simulink model "CombinedExperiment"  (R2020a)
settings: Solver=FixedStepAuto  StartTime=0.0  StopTime=tsim  FixedStep=baseRate  RelTol=1e-3  EnableMultiTasking=on
values from neighbouring files (symbols this model uses):
  baseRate = 0.1    [Run_Initializer.m]
  drop_states_BLACK = [1.36947387695313,1.22175756835938,-0.0161599479615688]    [Run_Initializer.m]
  drop_states_BLUE = [ xLength/2+0.9; yLength/2+0.5; 0]    [Run_Initializer.m]
  drop_states_RED = [ xLength/2+1.1; yLength/2; pi]    [Run_Initializer.m]
  F_thrusters_BLACK = 0.25.*ones(8,1)    [Run_Initializer.m]
  F_thrusters_BLUE = 0.25.*ones(8,1)    [Run_Initializer.m]
  F_thrusters_RED = 0.25.*ones(8,1)    [Run_Initializer.m]
  home_states_BLACK = [ xLength/2; yLength/2; 0]    [Run_Initializer.m]
  home_states_BLUE = [ xLength/2-0.9; yLength/2+0.5; 0]    [Run_Initializer.m]
  home_states_RED = [ xLength/2+1.1; yLength/2; pi]    [Run_Initializer.m]
  init_states_BLACK = [ xLength/2; yLength/2; 0]    [Run_Initializer.m]
  init_states_BLUE = [ xLength/2+0.9; yLength/2+0.5; 0]    [Run_Initializer.m]
  init_states_RED = [ xLength/2+1.1; yLength/2; pi]    [Run_Initializer.m]
  Kd_tb = 0.4    [Run_Initializer.m]
  Kd_tblue = 0.4    [Run_Initializer.m]
  Kd_tr = 0.4    [Run_Initializer.m]
  Kd_xb = 5    [Run_Initializer.m]
  Kd_xblue = 5    [Run_Initializer.m]
  Kd_xr = 5    [Run_Initializer.m]
  Kd_yb = 5    [Run_Initializer.m]
  Kd_yblue = 5    [Run_Initializer.m]
  Kd_yr = 5    [Run_Initializer.m]
  Kp_tb = 0.1    [Run_Initializer.m]
  Kp_tblue = 0.1    [Run_Initializer.m]
  Kp_tr = 0.1    [Run_Initializer.m]
  Kp_xb = 2    [Run_Initializer.m]
  Kp_xblue = 2    [Run_Initializer.m]
  Kp_xr = 2    [Run_Initializer.m]
  Kp_yb = 2    [Run_Initializer.m]
  Kp_yblue = 2    [Run_Initializer.m]
  Kp_yr = 2    [Run_Initializer.m]
  noise_variance_BLACK = 0    [Run_Initializer.m]
  noise_variance_BLUE = 0    [Run_Initializer.m]
  noise_variance_RED = 0    [Run_Initializer.m]
  Phase0_End = Phase0_Duration    (= 10)    [Run_Initializer.m]
  Phase1_End = Phase0_Duration + Phase1_Duration    (= 15)    [Run_Initializer.m]
  Phase2_End = Phase0_Duration + Phase1_Duration +                                   Phase2_Duration    (= 40)    [Run_Initializer.m]
  Phase3_End = Phase0_Duration + Phase1_Duration +                                   Phase2_Duration + Phase3_Duration    (= 117)    [Run_Initializer.m]
  Phase3_SubPhase1_End = Phase2_End + Phase3_SubPhase1_Duration    (= 41)    [Run_Initializer.m]
  Phase3_SubPhase2_End = Phase2_End + Phase3_SubPhase1_Duration +                                   Phase3_SubPhase2_Duration    (= 42)    [Run_Initializer.m]
  Phase3_SubPhase3_End = Phase2_End + Phase3_SubPhase1_Duration +                                   Phase3_SubPhase2_Duration +                                  Phase3_SubPhase3_Duration    (= 72)    [Run_Initializer.m]
  Phase3_SubPhase4_End = Phase2_End + Phase3_SubPhase1_Duration +                                   Phase3_SubPhase2_Duration +                                  Phase3_SubPhase3_Duration +                                  Phase3_SubPhase4_Duration    [Run_Initializer.m]
  Phase4_End = Phase0_Duration + Phase1_Duration +                                   Phase2_Duration + Phase3_Duration +                                   Phase4_Duration    (= 137)    [Run_Initializer.m]
  Phase5_End = Phase0_Duration + Phase1_Duration +                                   Phase2_Duration + Phase3_Duration +                                   Phase4_Duration + Phase5_Duration    (= 142)    [Run_Initializer.m]
  serverRate = 0.2    [Run_Initializer.m]
  thruster_dist2CG_BLACK = [83.42;-52.58;55.94;-60.05;54.08;-53.92;77.06;-55.94]    [Run_Initializer.m]
  thruster_dist2CG_BLUE = [83.42;-52.58;55.94;-60.05;54.08;-53.92;77.06;-55.94]    [Run_Initializer.m]
  thruster_dist2CG_RED = [49.92;-78.08;70.46;-63.54;81.08;-50.42;57.44;-75.96]    [Run_Initializer.m]
  xLength = 3.51155    [Run_Initializer.m]
  yLength = 2.41935    [Run_Initializer.m]
undefined symbols (not defined in the file or in its folder): DiscIntNeverNeededParam, platformSelection, simMode, WhoAmI
libraries: dspstat3 x18, raspberrypiBasiclib x10, dspsigops x9, embdlinuxlib x8, simulink x8, MainLibrary x5, mspfiltlib x3, dsparch4 x3, dspswit3 x2, sensehatlib x1
(part 9 of 9)

== matlab function CombinedExperiment/From Force//Torque to PWM Signal/Change BLACK Behavior/Calculate Thruster ON//OFF/Rotate Forces to Inertial/Create Rotation Matrix ==
  data: Rz input; C_Ib output
function C_Ib = RotateFrame(Rz)

C_bI = [  cos(Rz) sin(Rz)
         -sin(Rz) cos(Rz) ];

C_Ib = inv(C_bI);

end

== matlab function CombinedExperiment/From Force//Torque to PWM Signal/Change BLACK Behavior/Rotate Forces to Body/Create Rotation Matrix ==
  data: Rz input; C_bI output
function C_bI = RotateFrame(Rz)

C_bI = [  cos(Rz) sin(Rz)
         -sin(Rz) cos(Rz) ];

end

== matlab function CombinedExperiment/From Force//Torque to PWM Signal/Change RED Behavior/Calculate Thruster ON//OFF/MATLAB Function ==
  data: H output; thruster_dist2CG_RED parameter; F_thrusters_RED parameter
function H = MakeH(thruster_dist2CG_RED,F_thrusters_RED)

Vec1 = [ -1
         -1
          0 
          0
          1
          1
          0
          0 ];
      
Vec2 = [  0
          0
          1
          1
          0
          0
         -1
         -1 ];
     
Vec3 = thruster_dist2CG_RED./1000;

Mat1 = [Vec1, Vec2, Vec3]';

Mat2 = diag((F_thrusters_RED./2));

H    = Mat1*Mat2;

end

== matlab function CombinedExperiment/From Force//Torque to PWM Signal/Change RED Behavior/Calculate Thruster ON//OFF/MATLAB Function1 ==
  data: H output; thruster_dist2CG_RED parameter; F_thrusters_RED parameter
function H = MakeH(thruster_dist2CG_RED,F_thrusters_RED)

Vec1 = [ -1
         -1
          0 
          0
          1
          1
          0
          0 ];
      
Vec2 = [  0
          0
          1
          1
          0
          0
         -1
         -1 ];
     
Vec3 = thruster_dist2CG_RED./1000;

Mat1 = [Vec1, Vec2, Vec3]';

Mat2 = diag((F_thrusters_RED));

H    = Mat1*Mat2;

end

== matlab function CombinedExperiment/From Force//Torque to PWM Signal/Change RED Behavior/Calculate Thruster ON//OFF/MATLAB Function2 ==
  data: ThrustPer_Final output; ThrustPer input
function ThrustPer_Final  = ThrusterSat(ThrustPer)

ValveTime       = 0.007;
TControl        = 0.1;
ThrustPer_Final = zeros(8,1);

if max(ThrustPer) > 1
    ThrustPer_Sat = ThrustPer/max(ThrustPer);
else
    ThrustPer_Sat = ThrustPer;
end

for i = 1:8
    if ThrustPer_Sat(i) > ValveTime/TControl 
        ThrustPer_Final(i) = ThrustPer_Sat(i);
    else
        ThrustPer_Final(i) = 0;
    end
end
   

end

== matlab function CombinedExperiment/Simulate Plant Dynamics/RED Dynamics Model/MATLAB Function ==
  data: control_inputs input; x_ddot output; model_param parameter
function x_ddot = RED_dynamics(control_inputs, model_param)

%#codegen
% Fully define the size of x_ddot() for code generation:
x_ddot     = zeros(3,1);

% Extract the servicer model parameters from the model_param vector defined
% in initialize.m:
m_RED    = model_param(1);
I_RED    = model_param(2);

% Extract the control inputs from the control_input vector:
Fx        = control_inputs(1);              % [N]
Fy        = control_inputs(2);              % [N]
Tz        = control_inputs(3);              % [N.m]

% Calculate the state acceleration vector:
x_ddot(1) = Fx/m_RED;                      % [m/s^2]
x_ddot(2) = Fy/m_RED;                      % [m/s^2]
x_ddot(3) = Tz/I_RED;                      % [rad/s^2]

end

== matlab function CombinedExperiment/From Force//Torque to PWM Signal/Change RED Behavior/Calculate Thruster ON//OFF/Rotate Forces to Inertial/Create Rotation Matrix ==
  data: Rz input; C_Ib output
function C_Ib = RotateFrame(Rz)

C_bI = [  cos(Rz) sin(Rz)
         -sin(Rz) cos(Rz) ];

C_Ib = inv(C_bI);

end

== matlab function CombinedExperiment/Simulate Plant Dynamics/Sample and Hold Data to Match PhaseSpace (RED)/MATLAB Function ==
  data: TIME input; y output; SERVER input
function y = fcn(TIME, SERVER)

if mod(TIME,SERVER) == 0
    y = 1;
else
    y = 0;
end

== matlab function CombinedExperiment/Simulate Plant Dynamics/Sample and Hold Data to Match PhaseSpace (BLACK)/MATLAB Function ==
  data: TIME input; y output; SERVER input
function y = fcn(TIME, SERVER)

if mod(TIME,SERVER) == 0
    y = 1;
else
    y = 0;
end

== matlab function CombinedExperiment/From Force//Torque to PWM Signal/Change RED Behavior/Rotate Forces to Body/Create Rotation Matrix ==
  data: Rz input; C_bI output
function C_bI = RotateFrame(Rz)

C_bI = [  cos(Rz) sin(Rz)
         -sin(Rz) cos(Rz) ];

end

== matlab function CombinedExperiment/Phase #2: Move to Initial Position/Change RED Behavior/Hough Control/MATLAB Function2 ==
  data: Oy output; z input; Ox output
function [Oy, Ox]   = C3( z )
%C3 gives the rotation matrix about the z-axis for an angle 'z'
%   z - the angle about the z-axis which you rotate
%   A - the rotation matrix

Ox = [cos(z) sin(z); -sin(z) cos(z)]*[1;0];
Oy = [cos(z) sin(z); -sin(z) cos(z)]*[0;1];
end

== matlab function CombinedExperiment/Phase #2: Move to Initial Position/Change RED Behavior/Hough Control/MATLAB Function3 ==
  data: z input; Ox output
function Ox    = C3( z )
%C3 gives the rotation matrix about the z-axis for an angle 'z'
%   z - the angle about the z-axis which you rotate
%   A - the rotation matrix

Ox = [cos(z) sin(z); -sin(z) cos(z)]*[1;0];
end

== matlab function CombinedExperiment/Phase #2: Move to Initial Position/Change RED Behavior/Hough Control/MATLAB Function4 ==
  data: Oy input; e_out output; e_in input
function e_out = fcn(Oy, e_in)

a = sign(Oy'*e_in);
e_out = -a*norm(e_in);

== matlab function CombinedExperiment/Phase #3: Experiment/Change BLACK Behavior/Sub-Phase #4/Hough Control/MATLAB Function3 ==
  data: z input; Ox output
function Ox    = C3( z )
%C3 gives the rotation matrix about the z-axis for an angle 'z'
%   z - the angle about the z-axis which you rotate
%   A - the rotation matrix

Ox = [cos(z) sin(z); -sin(z) cos(z)]*[1;0];
end

== matlab function CombinedExperiment/Phase #4: Return Home/Change BLACK Behavior/Hough Control/MATLAB Function2 ==
  data: Oy output; z input; Ox output
function [Oy, Ox]   = C3( z )
%C3 gives the rotation matrix about the z-axis for an angle 'z'
%   z - the angle about the z-axis which you rotate
%   A - the rotation matrix

Ox = [cos(z) sin(z); -sin(z) cos(z)]*[1;0];
Oy = [cos(z) sin(z); -sin(z) cos(z)]*[0;1];
end

== matlab function CombinedExperiment/Phase #4: Return Home/Change BLACK Behavior/Hough Control/MATLAB Function3 ==
  data: z input; Ox output
function Ox    = C3( z )
%C3 gives the rotation matrix about the z-axis for an angle 'z'
%   z - the angle about the z-axis which you rotate
%   A - the rotation matrix

Ox = [cos(z) sin(z); -sin(z) cos(z)]*[1;0];
end

== matlab function CombinedExperiment/Simulate Plant Dynamics/BLACK Dynamics Model/MATLAB Function ==
  data: control_inputs input; x_ddot output; model_param parameter
function x_ddot = BLACK_dynamics(control_inputs, model_param)

%#codegen
% Fully define the size of x_ddot() for code generation:
x_ddot     = zeros(3,1);

% Extract the servicer model parameters from the model_param vector defined
% in initialize.m:
m_BLACK    = model_param(3);
I_BLACK    = model_param(4);

% Extract the control inputs from the control_input vector:
Fx        = control_inputs(1);              % [N]
Fy        = control_inputs(2);              % [N]
Tz        = control_inputs(3);              % [N.m]

% Calculate the state acceleration vector:
x_ddot(1) = Fx/m_BLACK;                      % [m/s^2]
x_ddot(2) = Fy/m_BLACK;                      % [m/s^2]
x_ddot(3) = Tz/I_BLACK;                      % [rad/s^2]

end

== matlab function CombinedExperiment/Phase #4: Return Home/Change BLACK Behavior/Hough Control/MATLAB Function4 ==
  data: Oy input; e_out output; e_in input
function e_out = fcn(Oy, e_in)

a = sign(Oy'*e_in);
e_out = -a*norm(e_in);

== matlab function CombinedExperiment/Phase #4: Return Home/Change RED Behavior/Hough Control/MATLAB Function2 ==
  data: Oy output; z input; Ox output
function [Oy, Ox]   = C3( z )
%C3 gives the rotation matrix about the z-axis for an angle 'z'
%   z - the angle about the z-axis which you rotate
%   A - the rotation matrix

Ox = [cos(z) sin(z); -sin(z) cos(z)]*[1;0];
Oy = [cos(z) sin(z); -sin(z) cos(z)]*[0;1];
end

== matlab function CombinedExperiment/Phase #4: Return Home/Change RED Behavior/Hough Control/MATLAB Function3 ==
  data: z input; Ox output
function Ox    = C3( z )
%C3 gives the rotation matrix about the z-axis for an angle 'z'
%   z - the angle about the z-axis which you rotate
%   A - the rotation matrix

Ox = [cos(z) sin(z); -sin(z) cos(z)]*[1;0];
end

== matlab function CombinedExperiment/Phase #4: Return Home/Change RED Behavior/Hough Control/MATLAB Function4 ==
  data: Oy input; e_out output; e_in input
function e_out = fcn(Oy, e_in)

a = sign(Oy'*e_in);
e_out = -a*norm(e_in);

== matlab function CombinedExperiment/Phase #2: Move to Initial Position/Change BLUE Behavior/Hough Control/MATLAB Function2 ==
  data: Oy output; z input; Ox output
function [Oy, Ox]   = C3( z )
%C3 gives the rotation matrix about the z-axis for an angle 'z'
%   z - the angle about the z-axis which you rotate
%   A - the rotation matrix

Ox = [cos(z) sin(z); -sin(z) cos(z)]*[1;0];
Oy = [cos(z) sin(z); -sin(z) cos(z)]*[0;1];
end

== matlab function CombinedExperiment/Phase #2: Move to Initial Position/Change BLUE Behavior/Hough Control/MATLAB Function3 ==
  data: z input; Ox output
function Ox    = C3( z )
%C3 gives the rotation matrix about the z-axis for an angle 'z'
%   z - the angle about the z-axis which you rotate
%   A - the rotation matrix

Ox = [cos(z) sin(z); -sin(z) cos(z)]*[1;0];
end

== matlab function CombinedExperiment/Phase #2: Move to Initial Position/Change BLUE Behavior/Hough Control/MATLAB Function4 ==
  data: Oy input; e_out output; e_in input
function e_out = fcn(Oy, e_in)

a = sign(Oy'*e_in);
e_out = -a*norm(e_in);

== matlab function CombinedExperiment/Phase #3: Experiment/Change BLUE Behavior/Sub-Phase #1/Hough Control/MATLAB Function2 ==
  data: Oy output; z input; Ox output
function [Oy, Ox]   = C3( z )
%C3 gives the rotation matrix about the z-axis for an angle 'z'
%   z - the angle about the z-axis which you rotate
%   A - the rotation matrix

Ox = [cos(z) sin(z); -sin(z) cos(z)]*[1;0];
Oy = [cos(z) sin(z); -sin(z) cos(z)]*[0;1];
end

== matlab function CombinedExperiment/Phase #3: Experiment/Change RED Behavior/Sub-Phase #4/Hough Control1/MATLAB Function2 ==
  data: Oy output; z input; Ox output
function [Oy, Ox]   = C3( z )
%C3 gives the rotation matrix about the z-axis for an angle 'z'
%   z - the angle about the z-axis which you rotate
%   A - the rotation matrix

Ox = [cos(z) sin(z); -sin(z) cos(z)]*[1;0];
Oy = [cos(z) sin(z); -sin(z) cos(z)]*[0;1];
end

== matlab function CombinedExperiment/Phase #3: Experiment/Change RED Behavior/Sub-Phase #4/Hough Control1/MATLAB Function3 ==
  data: z input; Ox output
function Ox    = C3( z )
%C3 gives the rotation matrix about the z-axis for an angle 'z'
%   z - the angle about the z-axis which you rotate
%   A - the rotation matrix

Ox = [cos(z) sin(z); -sin(z) cos(z)]*[1;0];
end

== matlab function CombinedExperiment/Phase #3: Experiment/Change RED Behavior/Sub-Phase #4/Hough Control1/MATLAB Function4 ==
  data: Oy input; e_out output; e_in input
function e_out = fcn(Oy, e_in)

a = sign(Oy'*e_in);
e_out = -a*norm(e_in);

== matlab function CombinedExperiment/Simulate Plant Dynamics/Sample and Hold Data to Match PhaseSpace (BLUE)/MATLAB Function ==
  data: TIME input; y output; SERVER input
function y = fcn(TIME, SERVER)

if mod(TIME,SERVER) == 0
    y = 1;
else
    y = 0;
end

== matlab function CombinedExperiment/Phase #3: Experiment/Change BLUE Behavior/Sub-Phase #1/Hough Control/MATLAB Function3 ==
  data: z input; Ox output
function Ox    = C3( z )
%C3 gives the rotation matrix about the z-axis for an angle 'z'
%   z - the angle about the z-axis which you rotate
%   A - the rotation matrix

Ox = [cos(z) sin(z); -sin(z) cos(z)]*[1;0];
end

== matlab function CombinedExperiment/Phase #3: Experiment/Change BLUE Behavior/Sub-Phase #1/Hough Control/MATLAB Function4 ==
  data: Oy input; e_out output; e_in input
function e_out = fcn(Oy, e_in)

a = sign(Oy'*e_in);
e_out = -a*norm(e_in);

== matlab function CombinedExperiment/Phase #3: Experiment/Change BLUE Behavior/Sub-Phase #4/Hough Control/MATLAB Function2 ==
  data: Oy output; z input; Ox output
function [Oy, Ox]   = C3( z )
%C3 gives the rotation matrix about the z-axis for an angle 'z'
%   z - the angle about the z-axis which you rotate
%   A - the rotation matrix

Ox = [cos(z) sin(z); -sin(z) cos(z)]*[1;0];
Oy = [cos(z) sin(z); -sin(z) cos(z)]*[0;1];
end

== matlab function CombinedExperiment/Phase #3: Experiment/Change RED Behavior/Sub-Phase #4/Hough Control/MATLAB Function2 ==
  data: Oy output; z input; Ox output
function [Oy, Ox]   = C3( z )
%C3 gives the rotation matrix about the z-axis for an angle 'z'
%   z - the angle about the z-axis which you rotate
%   A - the rotation matrix

Ox = [cos(z) sin(z); -sin(z) cos(z)]*[1;0];
Oy = [cos(z) sin(z); -sin(z) cos(z)]*[0;1];
end

== matlab function CombinedExperiment/Phase #3: Experiment/Change RED Behavior/Sub-Phase #4/Hough Control/MATLAB Function3 ==
  data: z input; Ox output
function Ox    = C3( z )
%C3 gives the rotation matrix about the z-axis for an angle 'z'
%   z - the angle about the z-axis which you rotate
%   A - the rotation matrix

Ox = [cos(z) sin(z); -sin(z) cos(z)]*[1;0];
end

== matlab function CombinedExperiment/Phase #3: Experiment/Change RED Behavior/Sub-Phase #4/Hough Control/MATLAB Function4 ==
  data: Oy input; e_out output; e_in input
function e_out = fcn(Oy, e_in)

a = sign(Oy'*e_in);
e_out = -a*norm(e_in);

== matlab function CombinedExperiment/Phase #3: Experiment/Change BLACK Behavior/Sub-Phase #4/Hough Control/MATLAB Function4 ==
  data: Oy input; e_out output; e_in input
function e_out = fcn(Oy, e_in)

a = sign(Oy'*e_in);
e_out = -a*norm(e_in);

== matlab function CombinedExperiment/Phase #3: Experiment/Change BLACK Behavior/Sub-Phase #1/Hough Control/MATLAB Function2 ==
  data: Oy output; z input; Ox output
function [Oy, Ox]   = C3( z )
%C3 gives the rotation matrix about the z-axis for an angle 'z'
%   z - the angle about the z-axis which you rotate
%   A - the rotation matrix

Ox = [cos(z) sin(z); -sin(z) cos(z)]*[1;0];
Oy = [cos(z) sin(z); -sin(z) cos(z)]*[0;1];
end

== matlab function CombinedExperiment/Phase #3: Experiment/Change BLACK Behavior/Sub-Phase #1/Hough Control/MATLAB Function3 ==
  data: z input; Ox output
function Ox    = C3( z )
%C3 gives the rotation matrix about the z-axis for an angle 'z'
%   z - the angle about the z-axis which you rotate
%   A - the rotation matrix

Ox = [cos(z) sin(z); -sin(z) cos(z)]*[1;0];
end

== matlab function CombinedExperiment/Phase #3: Experiment/Change BLACK Behavior/Sub-Phase #1/Hough Control/MATLAB Function4 ==
  data: Oy input; e_out output; e_in input
function e_out = fcn(Oy, e_in)

a = sign(Oy'*e_in);
e_out = -a*norm(e_in);

== matlab function CombinedExperiment/From Force//Torque to PWM Signal/Change BLUE Behavior/Calculate Thruster ON//OFF/MATLAB Function ==
  data: H output; thruster_dist2CG_BLUE parameter; F_thrusters_BLUE parameter
function H = MakeH(thruster_dist2CG_BLUE,F_thrusters_BLUE)

Vec1 = [ -1
         -1
          0 
          0
          1
          1
          0
          0 ];
      
Vec2 = [  0
          0
          1
          1
          0
          0
         -1
         -1 ];
     
Vec3 = thruster_dist2CG_BLUE./1000;

Mat1 = [Vec1, Vec2, Vec3]';

Mat2 = diag((F_thrusters_BLUE./2));

H    = Mat1*Mat2;

end

== matlab function CombinedExperiment/Phase #3: Experiment/Change BLUE Behavior/Sub-Phase #4/Hough Control/MATLAB Function3 ==
  data: z input; Ox output
function Ox    = C3( z )
%C3 gives the rotation matrix about the z-axis for an angle 'z'
%   z - the angle about the z-axis which you rotate
%   A - the rotation matrix

Ox = [cos(z) sin(z); -sin(z) cos(z)]*[1;0];
end

== matlab function CombinedExperiment/Phase #3: Experiment/Change BLUE Behavior/Sub-Phase #4/Hough Control/MATLAB Function4 ==
  data: Oy input; e_out output; e_in input
function e_out = fcn(Oy, e_in)

a = sign(Oy'*e_in);
e_out = -a*norm(e_in);

== matlab function CombinedExperiment/Phase #5: Hold Home/Change BLACK Behavior/Hough Control/MATLAB Function2 ==
  data: Oy output; z input; Ox output
function [Oy, Ox]   = C3( z )
%C3 gives the rotation matrix about the z-axis for an angle 'z'
%   z - the angle about the z-axis which you rotate
%   A - the rotation matrix

Ox = [cos(z) sin(z); -sin(z) cos(z)]*[1;0];
Oy = [cos(z) sin(z); -sin(z) cos(z)]*[0;1];
end

== matlab function CombinedExperiment/Phase #5: Hold Home/Change BLACK Behavior/Hough Control/MATLAB Function3 ==
  data: z input; Ox output
function Ox    = C3( z )
%C3 gives the rotation matrix about the z-axis for an angle 'z'
%   z - the angle about the z-axis which you rotate
%   A - the rotation matrix

Ox = [cos(z) sin(z); -sin(z) cos(z)]*[1;0];
end

== matlab function CombinedExperiment/Phase #5: Hold Home/Change BLACK Behavior/Hough Control/MATLAB Function4 ==
  data: Oy input; e_out output; e_in input
function e_out = fcn(Oy, e_in)

a = sign(Oy'*e_in);
e_out = -a*norm(e_in);

== matlab function CombinedExperiment/Phase #4: Return Home/Change BLUE Behavior/Hough Control/MATLAB Function2 ==
  data: Oy output; z input; Ox output
function [Oy, Ox]   = C3( z )
%C3 gives the rotation matrix about the z-axis for an angle 'z'
%   z - the angle about the z-axis which you rotate
%   A - the rotation matrix

Ox = [cos(z) sin(z); -sin(z) cos(z)]*[1;0];
Oy = [cos(z) sin(z); -sin(z) cos(z)]*[0;1];
end

== matlab function CombinedExperiment/Phase #4: Return Home/Change BLUE Behavior/Hough Control/MATLAB Function3 ==
  data: z input; Ox output
function Ox    = C3( z )
%C3 gives the rotation matrix about the z-axis for an angle 'z'
%   z - the angle about the z-axis which you rotate
%   A - the rotation matrix

Ox = [cos(z) sin(z); -sin(z) cos(z)]*[1;0];
end

== matlab function CombinedExperiment/Phase #4: Return Home/Change BLUE Behavior/Hough Control/MATLAB Function4 ==
  data: Oy input; e_out output; e_in input
function e_out = fcn(Oy, e_in)

a = sign(Oy'*e_in);
e_out = -a*norm(e_in);

== matlab function CombinedExperiment/Phase #5: Hold Home/Change RED Behavior/Hough Control/MATLAB Function2 ==
  data: Oy output; z input; Ox output
function [Oy, Ox]   = C3( z )
%C3 gives the rotation matrix about the z-axis for an angle 'z'
%   z - the angle about the z-axis which you rotate
%   A - the rotation matrix

Ox = [cos(z) sin(z); -sin(z) cos(z)]*[1;0];
Oy = [cos(z) sin(z); -sin(z) cos(z)]*[0;1];
end

== matlab function CombinedExperiment/Phase #5: Hold Home/Change RED Behavior/Hough Control/MATLAB Function3 ==
  data: z input; Ox output
function Ox    = C3( z )
%C3 gives the rotation matrix about the z-axis for an angle 'z'
%   z - the angle about the z-axis which you rotate
%   A - the rotation matrix

Ox = [cos(z) sin(z); -sin(z) cos(z)]*[1;0];
end

== matlab function CombinedExperiment/Phase #5: Hold Home/Change RED Behavior/Hough Control/MATLAB Function4 ==
  data: Oy input; e_out output; e_in input
function e_out = fcn(Oy, e_in)

a = sign(Oy'*e_in);
e_out = -a*norm(e_in);

== matlab function CombinedExperiment/From Force//Torque to PWM Signal/Change BLUE Behavior/Calculate Thruster ON//OFF/MATLAB Function1 ==
  data: H output; thruster_dist2CG_BLUE parameter; F_thrusters_BLUE parameter
function H = MakeH(thruster_dist2CG_BLUE,F_thrusters_BLUE)

Vec1 = [ -1
         -1
          0 
          0
          1
          1
          0
          0 ];
      
Vec2 = [  0
          0
          1
          1
          0
          0
         -1
         -1 ];
     
Vec3 = thruster_dist2CG_BLUE./1000;

Mat1 = [Vec1, Vec2, Vec3]';

Mat2 = diag((F_thrusters_BLUE./2));

H    = Mat1*Mat2;

end

== matlab function CombinedExperiment/Phase #5: Hold Home/Change BLUE Behavior/Hough Control/MATLAB Function2 ==
  data: Oy output; z input; Ox output
function [Oy, Ox]   = C3( z )
%C3 gives the rotation matrix about the z-axis for an angle 'z'
%   z - the angle about the z-axis which you rotate
%   A - the rotation matrix

Ox = [cos(z) sin(z); -sin(z) cos(z)]*[1;0];
Oy = [cos(z) sin(z); -sin(z) cos(z)]*[0;1];
end

== matlab function CombinedExperiment/Phase #5: Hold Home/Change BLUE Behavior/Hough Control/MATLAB Function3 ==
  data: z input; Ox output
function Ox    = C3( z )
%C3 gives the rotation matrix about the z-axis for an angle 'z'
%   z - the angle about the z-axis which you rotate
%   A - the rotation matrix

Ox = [cos(z) sin(z); -sin(z) cos(z)]*[1;0];
end

== matlab function CombinedExperiment/Phase #5: Hold Home/Change BLUE Behavior/Hough Control/MATLAB Function4 ==
  data: Oy input; e_out output; e_in input
function e_out = fcn(Oy, e_in)

a = sign(Oy'*e_in);
e_out = -a*norm(e_in);

== matlab function CombinedExperiment/From Torque, Command RW/Change RED Behavior/Calculate Saturated RPM Signal/Calculate RW RPM Increment ==
  data: Tz_Sat input; dRPM_RW output
function dRPM_RW = Calc_RW_RPM(Tz_Sat)

dRPM_RW =  (Tz_Sat/0.007244720)*(60/2/pi)*0.1;

end

== matlab function CombinedExperiment/From Torque, Command RW/Change RED Behavior/Wheel RPM to PWM/Check if RW is Ready ==
  data: Status input; EnableSig output; WheelRPM_In input; WheelRPM_Out output
function [EnableSig, WheelRPM_Out] = Check_Wheel_Status(Status, WheelRPM_In)

if Status == 0
    EnableSig    = 1;
    WheelRPM_Out = WheelRPM_In;
else
    EnableSig    = 0;
    WheelRPM_Out = 0;
end

end

== matlab function CombinedExperiment/From Torque, Command RW/Change RED Behavior/Wheel RPM to PWM/Get RW Direction ==
  data: MotorRPM_Sat input; WheelDirection output
function WheelDirection = GetDirection(MotorRPM_Sat)

if MotorRPM_Sat > 0
    WheelDirection = 0;
else
    WheelDirection = 1;
end
        
end

== matlab function CombinedExperiment/From Torque, Command RW/Change RED Behavior/Wheel RPM to PWM/RPM to PWM Value ==
  data: MotorRPM_Sat input; MotorPWM output
function MotorPWM = RPM2PWM(MotorRPM_Sat)

PWMRange = 0.9-0.1;

MotorPWM = ((MotorRPM_Sat*PWMRange)/7000) + 0.1;

end

== matlab function CombinedExperiment/Phase #3: Experiment/Change BLACK Behavior/Sub-Phase #4/BLACK_RzD1/Wrap1/MATLAB Function ==
  data: u input; wrappedAngle output
function wrappedAngle = wrapAngle(u)

wrappedAngle = atan2(sin(u),cos(u));

end

== matlab function CombinedExperiment/Gyroscope & Acceleration Algorithms/Change RED Behavior/Create Rotation Matrix ==
  data: Rz input; C_Ib output
function C_Ib = RotateFrame(Rz)

C_bI = [  cos(Rz) sin(Rz)
         -sin(Rz) cos(Rz) ];

C_Ib = inv(C_bI);

end

== matlab function CombinedExperiment/Gyroscope & Acceleration Algorithms/Change BLACK Behavior/Create Rotation Matrix ==
  data: Rz input; C_Ib output
function C_Ib = RotateFrame(Rz)

C_bI = [  cos(Rz) sin(Rz)
         -sin(Rz) cos(Rz) ];

C_Ib = inv(C_bI);

end

== matlab function CombinedExperiment/From Force//Torque to PWM Signal/Change BLUE Behavior/Calculate Thruster ON//OFF/MATLAB Function2 ==
  data: ThrustPer_Final output; ThrustPer input
function ThrustPer_Final  = ThrusterSat(ThrustPer)

ValveTime       = 0.007;
TControl        = 0.1;
ThrustPer_Final = zeros(8,1);

if max(ThrustPer) > 1
    ThrustPer_Sat = ThrustPer/max(ThrustPer);
else
    ThrustPer_Sat = ThrustPer;
end

for i = 1:8
    if ThrustPer_Sat(i) > ValveTime/TControl 
        ThrustPer_Final(i) = ThrustPer_Sat(i);
    else
        ThrustPer_Final(i) = 0;
    end
end
   

end

== matlab function CombinedExperiment/Gyroscope & Acceleration Algorithms/Change RED Behavior/ChangeOrientation ==
  data: u input; y output
function y = ChangeOrientation(u)

y = rotz(-90)*u';

== matlab function CombinedExperiment/Gyroscope & Acceleration Algorithms/Change BLACK Behavior/ChangeOrientation ==
  data: u input; y output
function y = ChangeOrientation(u)

y = rotz(-90)*u';

== matlab function CombinedExperiment/Gyroscope & Acceleration Algorithms/Change BLUE Behavior/ChangeOrientation ==
  data: u input; y output
function y = ChangeOrientation(u)

y = rotz(-90)*u';

== matlab function CombinedExperiment/Gyroscope & Acceleration Algorithms/Change BLUE Behavior/Create Rotation Matrix ==
  data: Rz input; C_Ib output
function C_Ib = RotateFrame(Rz)

C_bI = [  cos(Rz) sin(Rz)
         -sin(Rz) cos(Rz) ];

C_Ib = inv(C_bI);

end

== matlab function CombinedExperiment/From Force//Torque to PWM Signal/Change BLUE Behavior/Calculate Thruster ON//OFF/Rotate Forces to Inertial/Create Rotation Matrix ==
  data: Rz input; C_Ib output
function C_Ib = RotateFrame(Rz)

C_bI = [  cos(Rz) sin(Rz)
         -sin(Rz) cos(Rz) ];

C_Ib = inv(C_bI);

end

== matlab function CombinedExperiment/From Force//Torque to PWM Signal/Change BLUE Behavior/Rotate Forces to Body/Create Rotation Matrix ==
  data: Rz input; C_bI output
function C_bI = RotateFrame(Rz)

C_bI = [  cos(Rz) sin(Rz)
         -sin(Rz) cos(Rz) ];

end

== matlab function CombinedExperiment/Phase #2: Move to Initial Position/Change BLACK Behavior/Hough Control/MATLAB Function2 ==
  data: Oy output; z input; Ox output
function [Oy, Ox]   = C3( z )
%C3 gives the rotation matrix about the z-axis for an angle 'z'
%   z - the angle about the z-axis which you rotate
%   A - the rotation matrix

Ox = [cos(z) sin(z); -sin(z) cos(z)]*[1;0];
Oy = [cos(z) sin(z); -sin(z) cos(z)]*[0;1];
end

== matlab function CombinedExperiment/Phase #2: Move to Initial Position/Change BLACK Behavior/Hough Control/MATLAB Function3 ==
  data: z input; Ox output
function Ox    = C3( z )
%C3 gives the rotation matrix about the z-axis for an angle 'z'
%   z - the angle about the z-axis which you rotate
%   A - the rotation matrix

Ox = [cos(z) sin(z); -sin(z) cos(z)]*[1;0];
end

== matlab function CombinedExperiment/Simulate Plant Dynamics/BLUE  Dynamics Model/MATLAB Function ==
  data: control_inputs input; x_ddot output; model_param parameter
function x_ddot = BLUE_dynamics(control_inputs, model_param)

%#codegen
% Fully define the size of x_ddot() for code generation:
x_ddot     = zeros(3,1);

% Extract the servicer model parameters from the model_param vector defined
% in initialize.m:
m_BLUE    = model_param(5);
I_BLUE    = model_param(6);

% Extract the control inputs from the control_input vector:
Fx        = control_inputs(1);              % [N]
Fy        = control_inputs(2);              % [N]
Tz        = control_inputs(3);              % [N.m]

% Calculate the state acceleration vector:
x_ddot(1) = Fx/m_BLUE;                      % [m/s^2]
x_ddot(2) = Fy/m_BLUE;                      % [m/s^2]
x_ddot(3) = Tz/I_BLUE;                      % [rad/s^2]

end

== matlab function CombinedExperiment/Phase #2: Move to Initial Position/Change BLACK Behavior/Hough Control/MATLAB Function4 ==
  data: Oy input; e_out output; e_in input
function e_out = fcn(Oy, e_in)

a = sign(Oy'*e_in);
e_out = -a*norm(e_in);
